simulink model "LunarMicrogrid_Full_Arch"  (R2026b)
settings: Solver=ode23t  StopTime=simulation.timeSim  MaxStep=1/(5*solarPlant.converterSwitchingFrequency)  AbsTol=1e-3
PreLoadFcn:
  | run('LunarMicrogridA_Data');
values from neighbouring files (symbols this model uses):
  Csc = Csc_cell/Ns_sc*Np_sc    (= 200)    [LunarDAB_Params.m]
  eta_sc = 0.95    [LunarDAB_Params.m]
  fsw = 100e3    (= 100000)    [LunarDAB_Params.m]
  k_restore = 1    [LunarDAB_Params.m]
  kiCurrent = 2    [LunarDAB_Params.m]
  kiVoltage = 8    [LunarDAB_Params.m]
  kpCurrent = 0.005    [LunarDAB_Params.m]
  kpVoltage = 0.4    [LunarDAB_Params.m]
  lTotal = lSeries + Llk    [LunarDAB_Params.m]
  P170_dt = 1e-4    (= 0.0001)    [P170_PV_Initialize.m]
  P170_Imp = im(ix)    [P170_PV_Initialize.m]
  P170_Vmp = vm(ix)    [P170_PV_Initialize.m]
  Rd_bat = dV_droop/Ibat_max    (= 0.232258064516)    [LunarDAB_Params.m]
  SC_enable = 1    [LunarDAB_Params.m]
  thetaIC = 0    [LunarDAB_Params.m]
  thetaMaxDab = pi/4    (= 0.785398163397)    [LunarDAB_Params.m]
  Tsw = 1/fsw    (= 1e-05)    [LunarDAB_Params.m]
  Vsc0 = sqrt((Vsc_max^2 + Vsc_min^2)/2)    [LunarDAB_Params.m]
  Vsc_max = 119    [LunarDAB_Params.m]
  Vsc_min = 66    [LunarDAB_Params.m]
undefined symbols (not defined in the file or in its folder): a_lpf_sys, battery, bms, connectedLoad, dcVoltage, DiscIntNeverNeededParam, eta_dab, Ibat_sign, mmc, Ndab, P170_T, pvDroop, sc, sensor, socLimit, solarPlant
libraries: sl_discontinuities x13, fl_lib x13, nesl_utility x13, simulink x7, batteryecm_lib x1, simulink_extras x1, ee_lib x1
(part 8 of 8)

== system LunarMicrogrid_Full_Arch/Battery + DAB + Supercap/BESS Controller/PIctrl/Anti-windup/Disc. Clamping Ideal/Dead Zone ==
  preSat : Inport
  Upper Limit : Inport  Port=2  SampleTime=SampleTime
  Lower Limit : Inport  Port=3  SampleTime=SampleTime
  Disabled : Subsystem  VariantControl=Disabled
  Enabled : Subsystem  VariantControl=Enabled
  External : Subsystem  VariantControl=External
  DZ out : Outport

== system LunarMicrogrid_Full_Arch/Battery + DAB + Supercap/BESS Controller/PIctrl/Anti-windup/Disc. Clamping Parallel/Dead Zone ==
  preSat : Inport
  Upper Limit : Inport  Port=2  SampleTime=SampleTime
  Lower Limit : Inport  Port=3  SampleTime=SampleTime
  Disabled : Subsystem  VariantControl=Disabled
  Enabled : Subsystem  VariantControl=Enabled
  External : Subsystem  VariantControl=External
  DZ out : Outport

== system LunarMicrogrid_Full_Arch/Battery + DAB + Supercap/BESS Controller/PIctrl/Filter/Differentiator/Tsamp ==
  U : Inport  SampleTime=SampleTime
  Ts : Inport  Port=2  SampleTime=SampleTime
  External Ts : Subsystem  VariantControl=ExternalTs
  Internal Ts : Subsystem  VariantControl=InternalTs
  Out1 : Outport  SampleTime=SampleTime

== system LunarMicrogrid_Full_Arch/Battery + DAB + Supercap/BESS Controller/PIctrl/Filter/Disc. Backward Euler Filter/Tsamp ==
  N : Inport  SampleTime=SampleTime
  Ts : Inport  Port=2  SampleTime=SampleTime
  External Ts : Subsystem  VariantControl=ExternalTs
  Internal Ts : Subsystem  VariantControl=InternalTs
  Out1 : Outport  SampleTime=SampleTime

== system LunarMicrogrid_Full_Arch/Battery + DAB + Supercap/BESS Controller/PIctrl/Filter/Disc. Backward Euler Filter Only/Tsamp ==
  N : Inport  SampleTime=SampleTime
  Ts : Inport  Port=2  SampleTime=SampleTime
  External Ts : Subsystem  VariantControl=ExternalTs
  Internal Ts : Subsystem  VariantControl=InternalTs
  Out1 : Outport  SampleTime=SampleTime

== system LunarMicrogrid_Full_Arch/Battery + DAB + Supercap/BESS Controller/PIctrl/Filter/Disc. Trapezoidal Filter/Tsamp ==
  N : Inport  SampleTime=SampleTime
  Ts : Inport  Port=2  SampleTime=SampleTime
  External Ts : Subsystem  VariantControl=ExternalTs
  Internal Ts : Subsystem  VariantControl=InternalTs
  Out1 : Outport  SampleTime=SampleTime

== system LunarMicrogrid_Full_Arch/Battery + DAB + Supercap/BESS Controller/PIctrl/Filter/Disc. Trapezoidal Filter Only/Tsamp ==
  N : Inport  SampleTime=SampleTime
  Ts : Inport  Port=2  SampleTime=SampleTime
  External Ts : Subsystem  VariantControl=ExternalTs
  Internal Ts : Subsystem  VariantControl=InternalTs
  Out1 : Outport  SampleTime=SampleTime

== system LunarMicrogrid_Full_Arch/Battery + DAB + Supercap/BESS Controller/DABCtrl2/Anti-windup/Cont. Clamping Ideal/Dead Zone/Disabled ==

== system LunarMicrogrid_Full_Arch/Battery + DAB + Supercap/BESS Controller/DABCtrl2/Anti-windup/Cont. Clamping Ideal/Dead Zone/Enabled ==
  preSat : Inport
  DeadZone : DeadZone  DisableCoverage=on  LowerValue=LowerSaturationLimit  UpperValue=UpperSaturationLimit  LinearizeAsGain=off  SaturateOnIntegerOverflow=off
  DZ out : Outport
  wires:
  preSat/1 -> DeadZone/1
  DeadZone/1 -> DZ out/1

== system LunarMicrogrid_Full_Arch/Battery + DAB + Supercap/BESS Controller/DABCtrl2/Anti-windup/Cont. Clamping Ideal/Dead Zone/External ==
  preSat : Inport
  Upper Limit : Inport  Port=2  SampleTime=SampleTime
  Lower Limit : Inport  Port=3  SampleTime=SampleTime
  Dead Zone Dynamic1 : sl_discontinuities/Dead Zone Dynamic
  DZ out : Outport
  wires:
  preSat/1 -> Dead Zone Dynamic1/2
  Lower Limit/1 -> Dead Zone Dynamic1/3
  Upper Limit/1 -> Dead Zone Dynamic1/1
  Dead Zone Dynamic1/1 -> DZ out/1

== system LunarMicrogrid_Full_Arch/Battery + DAB + Supercap/BESS Controller/DABCtrl2/Anti-windup/Cont. Clamping Parallel/Dead Zone/Disabled ==

== system LunarMicrogrid_Full_Arch/Battery + DAB + Supercap/BESS Controller/DABCtrl2/Anti-windup/Cont. Clamping Parallel/Dead Zone/Enabled ==
  preSat : Inport
  DeadZone : DeadZone  DisableCoverage=on  LowerValue=LowerSaturationLimit  UpperValue=UpperSaturationLimit  LinearizeAsGain=off  SaturateOnIntegerOverflow=off
  DZ out : Outport
  wires:
  preSat/1 -> DeadZone/1
  DeadZone/1 -> DZ out/1

== system LunarMicrogrid_Full_Arch/Battery + DAB + Supercap/BESS Controller/DABCtrl2/Anti-windup/Cont. Clamping Parallel/Dead Zone/External ==
  preSat : Inport
  Upper Limit : Inport  Port=2  SampleTime=SampleTime
  Lower Limit : Inport  Port=3  SampleTime=SampleTime
  Dead Zone Dynamic : sl_discontinuities/Dead Zone Dynamic
  DZ out : Outport
  wires:
  preSat/1 -> Dead Zone Dynamic/2
  Lower Limit/1 -> Dead Zone Dynamic/3
  Upper Limit/1 -> Dead Zone Dynamic/1
  Dead Zone Dynamic/1 -> DZ out/1

== system LunarMicrogrid_Full_Arch/Battery + DAB + Supercap/BESS Controller/DABCtrl2/Anti-windup/Disc. Clamping Ideal/Dead Zone/Disabled ==

== system LunarMicrogrid_Full_Arch/Battery + DAB + Supercap/BESS Controller/DABCtrl2/Anti-windup/Disc. Clamping Ideal/Dead Zone/Enabled ==
  preSat : Inport
  DeadZone : DeadZone  DisableCoverage=on  LowerValue=LowerSaturationLimit  UpperValue=UpperSaturationLimit  LinearizeAsGain=off  SaturateOnIntegerOverflow=off
  DZ out : Outport
  wires:
  DeadZone/1 -> DZ out/1
  preSat/1 -> DeadZone/1

== system LunarMicrogrid_Full_Arch/Battery + DAB + Supercap/BESS Controller/DABCtrl2/Anti-windup/Disc. Clamping Ideal/Dead Zone/External ==
  preSat : Inport
  Upper Limit : Inport  Port=2  SampleTime=SampleTime
  Lower Limit : Inport  Port=3  SampleTime=SampleTime
  Dead Zone Dynamic : sl_discontinuities/Dead Zone Dynamic
  DZ out : Outport
  wires:
  Dead Zone Dynamic/1 -> DZ out/1
  Upper Limit/1 -> Dead Zone Dynamic/1
  Lower Limit/1 -> Dead Zone Dynamic/3
  preSat/1 -> Dead Zone Dynamic/2

== system LunarMicrogrid_Full_Arch/Battery + DAB + Supercap/BESS Controller/DABCtrl2/Anti-windup/Disc. Clamping Parallel/Dead Zone/Disabled ==

== system LunarMicrogrid_Full_Arch/Battery + DAB + Supercap/BESS Controller/DABCtrl2/Anti-windup/Disc. Clamping Parallel/Dead Zone/Enabled ==
  preSat : Inport
  DeadZone : DeadZone  DisableCoverage=on  LowerValue=LowerSaturationLimit  UpperValue=UpperSaturationLimit  LinearizeAsGain=off  SaturateOnIntegerOverflow=off
  DZ out : Outport
  wires:
  DeadZone/1 -> DZ out/1
  preSat/1 -> DeadZone/1

== system LunarMicrogrid_Full_Arch/Battery + DAB + Supercap/BESS Controller/DABCtrl2/Anti-windup/Disc. Clamping Parallel/Dead Zone/External ==
  preSat : Inport
  Upper Limit : Inport  Port=2  SampleTime=SampleTime
  Lower Limit : Inport  Port=3  SampleTime=SampleTime
  Dead Zone Dynamic : sl_discontinuities/Dead Zone Dynamic
  DZ out : Outport
  wires:
  Dead Zone Dynamic/1 -> DZ out/1
  Upper Limit/1 -> Dead Zone Dynamic/1
  Lower Limit/1 -> Dead Zone Dynamic/3
  preSat/1 -> Dead Zone Dynamic/2

== system LunarMicrogrid_Full_Arch/Battery + DAB + Supercap/BESS Controller/DABCtrl2/Filter/Differentiator/Tsamp/External Ts ==
  U : Inport  SampleTime=SampleTime
  Ts : Inport  Port=2  SampleTime=SampleTime
  Udiff*Ts Prod Out : Product  Inputs=*/  OutMin=UdiffTsProdOutMin  OutMax=UdiffTsProdOutMax  RndMeth=Simplest  SampleTime=SampleTime
  Out1 : Outport  SampleTime=SampleTime
  wires:
  U/1 -> Udiff*Ts Prod Out/1
  Udiff*Ts Prod Out/1 -> Out1/1
  Ts/1 -> Udiff*Ts Prod Out/2

== system LunarMicrogrid_Full_Arch/Battery + DAB + Supercap/BESS Controller/DABCtrl2/Filter/Differentiator/Tsamp/Internal Ts ==
  U : Inport  SampleTime=SampleTime
  Ts : Inport  Port=2  SampleTime=SampleTime
  Terminator : Terminator
  Tsamp : SampleTimeMath  TsampMathOp=/  TsampMathImp=Offline Scaling Adjustment  RndMeth=Simplest
  Out1 : Outport  SampleTime=SampleTime
  wires:
  U/1 -> Tsamp/1
  Ts/1 -> Terminator/1
  Tsamp/1 -> Out1/1

== system LunarMicrogrid_Full_Arch/Battery + DAB + Supercap/BESS Controller/DABCtrl2/Filter/Disc. Backward Euler Filter/Tsamp/External Ts ==
  N : Inport  SampleTime=SampleTime
  Ts : Inport  Port=2  SampleTime=SampleTime
  N*Ts Prod Out : Product  OutMin=NTsProdOutMin  OutMax=NTsProdOutMax  RndMeth=Simplest  SampleTime=SampleTime
  Out1 : Outport  SampleTime=SampleTime
  wires:
  Ts/1 -> N*Ts Prod Out/2
  N*Ts Prod Out/1 -> Out1/1
  N/1 -> N*Ts Prod Out/1

== system LunarMicrogrid_Full_Arch/Battery + DAB + Supercap/BESS Controller/DABCtrl2/Filter/Disc. Backward Euler Filter/Tsamp/Internal Ts ==
  N : Inport  SampleTime=SampleTime
  Ts : Inport  Port=2  SampleTime=SampleTime
  Terminator : Terminator
  Tsamp : SampleTimeMath  TsampMathOp=*  RndMeth=Simplest
  Out1 : Outport  SampleTime=SampleTime
  wires:
  Tsamp/1 -> Out1/1
  Ts/1 -> Terminator/1
  N/1 -> Tsamp/1

== system LunarMicrogrid_Full_Arch/Battery + DAB + Supercap/BESS Controller/DABCtrl2/Filter/Disc. Backward Euler Filter Only/Tsamp/External Ts ==
  N : Inport  SampleTime=SampleTime
  Ts : Inport  Port=2  SampleTime=SampleTime
  N*Ts Prod Out : Product  OutMin=NTsProdOutMin  OutMax=NTsProdOutMax  SampleTime=SampleTime
  Out1 : Outport  SampleTime=SampleTime
  wires:
  N/1 -> N*Ts Prod Out/1
  N*Ts Prod Out/1 -> Out1/1
  Ts/1 -> N*Ts Prod Out/2

== system LunarMicrogrid_Full_Arch/Battery + DAB + Supercap/BESS Controller/DABCtrl2/Filter/Disc. Backward Euler Filter Only/Tsamp/Internal Ts ==
  N : Inport  SampleTime=SampleTime
  Ts : Inport  Port=2  SampleTime=SampleTime
  Terminator : Terminator
  Tsamp : SampleTimeMath  TsampMathOp=*
  Out1 : Outport  SampleTime=SampleTime
  wires:
  N/1 -> Tsamp/1
  Ts/1 -> Terminator/1
  Tsamp/1 -> Out1/1

== system LunarMicrogrid_Full_Arch/Battery + DAB + Supercap/BESS Controller/DABCtrl2/Filter/Disc. Trapezoidal Filter/Tsamp/External Ts ==
  N : Inport  SampleTime=SampleTime
  Ts : Inport  Port=2  SampleTime=SampleTime
  Gain : Gain  Gain=0.5  RndMeth=Simplest
  N*Ts Prod Out : Product  OutMin=NTsProdOutMin  OutMax=NTsProdOutMax  RndMeth=Simplest  SampleTime=SampleTime
  Out1 : Outport  SampleTime=SampleTime
  wires:
  Gain/1 -> N*Ts Prod Out/2
  Ts/1 -> Gain/1
  N*Ts Prod Out/1 -> Out1/1
  N/1 -> N*Ts Prod Out/1

== system LunarMicrogrid_Full_Arch/Battery + DAB + Supercap/BESS Controller/DABCtrl2/Filter/Disc. Trapezoidal Filter/Tsamp/Internal Ts ==
  N : Inport  SampleTime=SampleTime
  Ts : Inport  Port=2  SampleTime=SampleTime
  Terminator : Terminator
  Tsamp : SampleTimeMath  TsampMathOp=*  weightValue=0.5  RndMeth=Simplest
  Out1 : Outport  SampleTime=SampleTime
  wires:
  Tsamp/1 -> Out1/1
  Ts/1 -> Terminator/1
  N/1 -> Tsamp/1

== system LunarMicrogrid_Full_Arch/Battery + DAB + Supercap/BESS Controller/DABCtrl2/Filter/Disc. Trapezoidal Filter Only/Tsamp/External Ts ==
  N : Inport  SampleTime=SampleTime
  Ts : Inport  Port=2  SampleTime=SampleTime
  Gain : Gain  Gain=0.5
  N*Ts Prod Out : Product  OutMin=NTsProdOutMin  OutMax=NTsProdOutMax  SampleTime=SampleTime
  Out1 : Outport  SampleTime=SampleTime
  wires:
  N/1 -> N*Ts Prod Out/1
  N*Ts Prod Out/1 -> Out1/1
  Ts/1 -> Gain/1
  Gain/1 -> N*Ts Prod Out/2

== system LunarMicrogrid_Full_Arch/Battery + DAB + Supercap/BESS Controller/DABCtrl2/Filter/Disc. Trapezoidal Filter Only/Tsamp/Internal Ts ==
  N : Inport  SampleTime=SampleTime
  Ts : Inport  Port=2  SampleTime=SampleTime
  Terminator : Terminator
  Tsamp : SampleTimeMath  TsampMathOp=*  weightValue=0.5
  Out1 : Outport  SampleTime=SampleTime
  wires:
  N/1 -> Tsamp/1
  Ts/1 -> Terminator/1
  Tsamp/1 -> Out1/1

== system LunarMicrogrid_Full_Arch/Battery + DAB + Supercap/BESS Controller/PIctrl/Anti-windup/Cont. Clamping Ideal/Dead Zone/Disabled ==

== system LunarMicrogrid_Full_Arch/Battery + DAB + Supercap/BESS Controller/PIctrl/Anti-windup/Cont. Clamping Ideal/Dead Zone/Enabled ==
  preSat : Inport
  DeadZone : DeadZone  DisableCoverage=on  LowerValue=LowerSaturationLimit  UpperValue=UpperSaturationLimit  LinearizeAsGain=off  SaturateOnIntegerOverflow=off
  DZ out : Outport
  wires:
  preSat/1 -> DeadZone/1
  DeadZone/1 -> DZ out/1

== system LunarMicrogrid_Full_Arch/Battery + DAB + Supercap/BESS Controller/PIctrl/Anti-windup/Cont. Clamping Ideal/Dead Zone/External ==
  preSat : Inport
  Upper Limit : Inport  Port=2  SampleTime=SampleTime
  Lower Limit : Inport  Port=3  SampleTime=SampleTime
  Dead Zone Dynamic1 : sl_discontinuities/Dead Zone Dynamic
  DZ out : Outport
  wires:
  preSat/1 -> Dead Zone Dynamic1/2
  Lower Limit/1 -> Dead Zone Dynamic1/3
  Upper Limit/1 -> Dead Zone Dynamic1/1
  Dead Zone Dynamic1/1 -> DZ out/1

== system LunarMicrogrid_Full_Arch/Battery + DAB + Supercap/BESS Controller/PIctrl/Anti-windup/Cont. Clamping Parallel/Dead Zone/Disabled ==

== system LunarMicrogrid_Full_Arch/Battery + DAB + Supercap/BESS Controller/PIctrl/Anti-windup/Cont. Clamping Parallel/Dead Zone/Enabled ==
  preSat : Inport
  DeadZone : DeadZone  DisableCoverage=on  LowerValue=LowerSaturationLimit  UpperValue=UpperSaturationLimit  LinearizeAsGain=off  SaturateOnIntegerOverflow=off
  DZ out : Outport
  wires:
  preSat/1 -> DeadZone/1
  DeadZone/1 -> DZ out/1

== system LunarMicrogrid_Full_Arch/Battery + DAB + Supercap/BESS Controller/PIctrl/Anti-windup/Cont. Clamping Parallel/Dead Zone/External ==
  preSat : Inport
  Upper Limit : Inport  Port=2  SampleTime=SampleTime
  Lower Limit : Inport  Port=3  SampleTime=SampleTime
  Dead Zone Dynamic : sl_discontinuities/Dead Zone Dynamic
  DZ out : Outport
  wires:
  preSat/1 -> Dead Zone Dynamic/2
  Lower Limit/1 -> Dead Zone Dynamic/3
  Upper Limit/1 -> Dead Zone Dynamic/1
  Dead Zone Dynamic/1 -> DZ out/1

== system LunarMicrogrid_Full_Arch/Battery + DAB + Supercap/BESS Controller/PIctrl/Anti-windup/Disc. Clamping Ideal/Dead Zone/Disabled ==

== system LunarMicrogrid_Full_Arch/Battery + DAB + Supercap/BESS Controller/PIctrl/Anti-windup/Disc. Clamping Ideal/Dead Zone/Enabled ==
  preSat : Inport
  DeadZone : DeadZone  DisableCoverage=on  LowerValue=LowerSaturationLimit  UpperValue=UpperSaturationLimit  LinearizeAsGain=off  SaturateOnIntegerOverflow=off
  DZ out : Outport
  wires:
  DeadZone/1 -> DZ out/1
  preSat/1 -> DeadZone/1

== system LunarMicrogrid_Full_Arch/Battery + DAB + Supercap/BESS Controller/PIctrl/Anti-windup/Disc. Clamping Ideal/Dead Zone/External ==
  preSat : Inport
  Upper Limit : Inport  Port=2  SampleTime=SampleTime
  Lower Limit : Inport  Port=3  SampleTime=SampleTime
  Dead Zone Dynamic : sl_discontinuities/Dead Zone Dynamic
  DZ out : Outport
  wires:
  Dead Zone Dynamic/1 -> DZ out/1
  Upper Limit/1 -> Dead Zone Dynamic/1
  Lower Limit/1 -> Dead Zone Dynamic/3
  preSat/1 -> Dead Zone Dynamic/2

== system LunarMicrogrid_Full_Arch/Battery + DAB + Supercap/BESS Controller/PIctrl/Anti-windup/Disc. Clamping Parallel/Dead Zone/Disabled ==

== system LunarMicrogrid_Full_Arch/Battery + DAB + Supercap/BESS Controller/PIctrl/Anti-windup/Disc. Clamping Parallel/Dead Zone/Enabled ==
  preSat : Inport
  DeadZone : DeadZone  DisableCoverage=on  LowerValue=LowerSaturationLimit  UpperValue=UpperSaturationLimit  LinearizeAsGain=off  SaturateOnIntegerOverflow=off
  DZ out : Outport
  wires:
  DeadZone/1 -> DZ out/1
  preSat/1 -> DeadZone/1

== system LunarMicrogrid_Full_Arch/Battery + DAB + Supercap/BESS Controller/PIctrl/Anti-windup/Disc. Clamping Parallel/Dead Zone/External ==
  preSat : Inport
  Upper Limit : Inport  Port=2  SampleTime=SampleTime
  Lower Limit : Inport  Port=3  SampleTime=SampleTime
  Dead Zone Dynamic : sl_discontinuities/Dead Zone Dynamic
  DZ out : Outport
  wires:
  Dead Zone Dynamic/1 -> DZ out/1
  Upper Limit/1 -> Dead Zone Dynamic/1
  Lower Limit/1 -> Dead Zone Dynamic/3
  preSat/1 -> Dead Zone Dynamic/2

== system LunarMicrogrid_Full_Arch/Battery + DAB + Supercap/BESS Controller/PIctrl/Filter/Differentiator/Tsamp/External Ts ==
  U : Inport  SampleTime=SampleTime
  Ts : Inport  Port=2  SampleTime=SampleTime
  Udiff*Ts Prod Out : Product  Inputs=*/  OutMin=UdiffTsProdOutMin  OutMax=UdiffTsProdOutMax  RndMeth=Simplest  SampleTime=SampleTime
  Out1 : Outport  SampleTime=SampleTime
  wires:
  U/1 -> Udiff*Ts Prod Out/1
  Udiff*Ts Prod Out/1 -> Out1/1
  Ts/1 -> Udiff*Ts Prod Out/2

== system LunarMicrogrid_Full_Arch/Battery + DAB + Supercap/BESS Controller/PIctrl/Filter/Differentiator/Tsamp/Internal Ts ==
  U : Inport  SampleTime=SampleTime
  Ts : Inport  Port=2  SampleTime=SampleTime
  Terminator : Terminator
  Tsamp : SampleTimeMath  TsampMathOp=/  TsampMathImp=Offline Scaling Adjustment  RndMeth=Simplest
  Out1 : Outport  SampleTime=SampleTime
  wires:
  U/1 -> Tsamp/1
  Ts/1 -> Terminator/1
  Tsamp/1 -> Out1/1

== system LunarMicrogrid_Full_Arch/Battery + DAB + Supercap/BESS Controller/PIctrl/Filter/Disc. Backward Euler Filter/Tsamp/External Ts ==
  N : Inport  SampleTime=SampleTime
  Ts : Inport  Port=2  SampleTime=SampleTime
  N*Ts Prod Out : Product  OutMin=NTsProdOutMin  OutMax=NTsProdOutMax  RndMeth=Simplest  SampleTime=SampleTime
  Out1 : Outport  SampleTime=SampleTime
  wires:
  Ts/1 -> N*Ts Prod Out/2
  N*Ts Prod Out/1 -> Out1/1
  N/1 -> N*Ts Prod Out/1

== system LunarMicrogrid_Full_Arch/Battery + DAB + Supercap/BESS Controller/PIctrl/Filter/Disc. Backward Euler Filter/Tsamp/Internal Ts ==
  N : Inport  SampleTime=SampleTime
  Ts : Inport  Port=2  SampleTime=SampleTime
  Terminator : Terminator
  Tsamp : SampleTimeMath  TsampMathOp=*  RndMeth=Simplest
  Out1 : Outport  SampleTime=SampleTime
  wires:
  Tsamp/1 -> Out1/1
  Ts/1 -> Terminator/1
  N/1 -> Tsamp/1

== system LunarMicrogrid_Full_Arch/Battery + DAB + Supercap/BESS Controller/PIctrl/Filter/Disc. Backward Euler Filter Only/Tsamp/External Ts ==
  N : Inport  SampleTime=SampleTime
  Ts : Inport  Port=2  SampleTime=SampleTime
  N*Ts Prod Out : Product  OutMin=NTsProdOutMin  OutMax=NTsProdOutMax  SampleTime=SampleTime
  Out1 : Outport  SampleTime=SampleTime
  wires:
  N/1 -> N*Ts Prod Out/1
  N*Ts Prod Out/1 -> Out1/1
  Ts/1 -> N*Ts Prod Out/2

== system LunarMicrogrid_Full_Arch/Battery + DAB + Supercap/BESS Controller/PIctrl/Filter/Disc. Backward Euler Filter Only/Tsamp/Internal Ts ==
  N : Inport  SampleTime=SampleTime
  Ts : Inport  Port=2  SampleTime=SampleTime
  Terminator : Terminator
  Tsamp : SampleTimeMath  TsampMathOp=*
  Out1 : Outport  SampleTime=SampleTime
  wires:
  N/1 -> Tsamp/1
  Ts/1 -> Terminator/1
  Tsamp/1 -> Out1/1

== system LunarMicrogrid_Full_Arch/Battery + DAB + Supercap/BESS Controller/PIctrl/Filter/Disc. Trapezoidal Filter/Tsamp/External Ts ==
  N : Inport  SampleTime=SampleTime
  Ts : Inport  Port=2  SampleTime=SampleTime
  Gain : Gain  Gain=0.5  RndMeth=Simplest
  N*Ts Prod Out : Product  OutMin=NTsProdOutMin  OutMax=NTsProdOutMax  RndMeth=Simplest  SampleTime=SampleTime
  Out1 : Outport  SampleTime=SampleTime
  wires:
  Gain/1 -> N*Ts Prod Out/2
  Ts/1 -> Gain/1
  N*Ts Prod Out/1 -> Out1/1
  N/1 -> N*Ts Prod Out/1

== system LunarMicrogrid_Full_Arch/Battery + DAB + Supercap/BESS Controller/PIctrl/Filter/Disc. Trapezoidal Filter/Tsamp/Internal Ts ==
  N : Inport  SampleTime=SampleTime
  Ts : Inport  Port=2  SampleTime=SampleTime
  Terminator : Terminator
  Tsamp : SampleTimeMath  TsampMathOp=*  weightValue=0.5  RndMeth=Simplest
  Out1 : Outport  SampleTime=SampleTime
  wires:
  Tsamp/1 -> Out1/1
  Ts/1 -> Terminator/1
  N/1 -> Tsamp/1

== system LunarMicrogrid_Full_Arch/Battery + DAB + Supercap/BESS Controller/PIctrl/Filter/Disc. Trapezoidal Filter Only/Tsamp/External Ts ==
  N : Inport  SampleTime=SampleTime
  Ts : Inport  Port=2  SampleTime=SampleTime
  Gain : Gain  Gain=0.5
  N*Ts Prod Out : Product  OutMin=NTsProdOutMin  OutMax=NTsProdOutMax  SampleTime=SampleTime
  Out1 : Outport  SampleTime=SampleTime
  wires:
  N/1 -> N*Ts Prod Out/1
  N*Ts Prod Out/1 -> Out1/1
  Ts/1 -> Gain/1
  Gain/1 -> N*Ts Prod Out/2

== system LunarMicrogrid_Full_Arch/Battery + DAB + Supercap/BESS Controller/PIctrl/Filter/Disc. Trapezoidal Filter Only/Tsamp/Internal Ts ==
  N : Inport  SampleTime=SampleTime
  Ts : Inport  Port=2  SampleTime=SampleTime
  Terminator : Terminator
  Tsamp : SampleTimeMath  TsampMathOp=*  weightValue=0.5
  Out1 : Outport  SampleTime=SampleTime
  wires:
  N/1 -> Tsamp/1
  Ts/1 -> Terminator/1
  Tsamp/1 -> Out1/1

== matlab function LunarMicrogrid_Full_Arch/MMC Intertie to Site B (1.5 kV)/MMC Intertie ==
  settings: updateMethod=DISCRETE  sampleTime=mmc.dt
  data: Vbus input; I_LV output; P_rx input; P output; V_HV output; I_line output; V_rx output; phi output; mmc parameter
function [I_LV, P, V_HV, I_line, V_rx, phi] = fcn(Vbus, P_rx, mmc)
% averaged MMC intertie, same equations as mmc_and_bus_current.m
% uses the real 120 V bus voltage instead of a fixed 120 V
persistent V I Vrx z
if isempty(V)
    V = mmc.V0; I = mmc.I0; Vrx = mmc.Vrx0; z = mmc.z0;
end
dt = mmc.dt;
vb = max(Vbus, 1);
e = mmc.V_ref - V;
u = mmc.Kp*e + mmc.Ki*z;
phi = min(max(u, -pi/2), pi/2);
if ~((u >= pi/2 && e > 0) || (u <= -pi/2 && e < 0)), z = z + e*dt; end
Kc = mmc.n*vb*V/(2*pi*mmc.rv*mmc.f*mmc.Lleak);
P = mmc.Npar*Kc*phi*(1 - abs(phi)/pi);
dV  = (P/V - I)/mmc.C_HV;
dI  = (V - Vrx - mmc.R_line*I)/mmc.L_line;
dVr = (I - P_rx/max(Vrx, 1))/mmc.C_RX;
V_HV = V; I_line = I; V_rx = Vrx;
V = V + dV*dt; I = I + dI*dt; Vrx = Vrx + dVr*dt;
I_LV = P/vb;
end

== matlab function LunarMicrogrid_Full_Arch/PV Array + Converter/PV_MPPT_6module ==
  settings: updateMethod=DISCRETE  sampleTime=P170_dt
  data: G input; Ibus output; T input; Vbus input; en input; VmpT input; ImpT input; Pbus output; Pavail output; Vpv output; Ipv output; Imod output; duty output
function [Ibus, Pbus, Pavail, Vpv, Ipv, Imod, duty] = fcn(G,T,Vbus,en,VmpT,ImpT)
%#codegen
% EOL teammate MPP data; illustrative piecewise I-V fit.
% Shared PV bus, single coordinated P&O, six averaged PI branches.
persistent Vcmd dir Pprev count il integ
if isempty(Vcmd)
 Vcmd=217; dir=1; Pprev=0; count=0; il=zeros(6,1); integ=zeros(6,1);
end
dt=1e-4; eta=0.96; Gref=1367;
gs=max(0,min(1.5,G/Gref));
vmp=max(10,VmpT); imp=max(0,ImpT)*gs;
% Curve passes through Isc, Imp at Vmp, and zero at Voc.
% Isc=1.04 Imp, Voc=1.13 Vmp are MODEL ASSUMPTIONS.
isc=1.04*imp; voc=1.13*vmp;
Vcmd=max(0.5*vmp,min(0.99*voc,Vcmd));
if Vcmd<=vmp
 ipv=max(0,isc-(isc-imp)*(Vcmd/vmp)^2);
else
 ipv=max(0,imp*(voc-Vcmd)/(voc-vmp));
end
Ppv=Vcmd*ipv; Pavail=max(0,vmp*imp*eta);
count=count+1;
if count>=100
 if Ppv<Pprev, dir=-dir; end
 Vcmd=Vcmd+dir*0.5; Pprev=Ppv; count=0;
end
% Power-to-current reference; current limited by PV production.
v=max(30,Vbus);
Ptarget=max(0,min(Ppv*eta,Pavail))*max(0,min(1,en));
Iref=Ptarget/v/6;
Imod=zeros(6,1); duty=zeros(6,1);
for k=1:6
 % Averaged current PI with feedforward; shared-array duty proxy.
 err=Iref-il(k);
 dff=Vbus/max(1,1.15*Vcmd);
 d=max(0,min(0.85,dff+0.0015*err+integ(k)));
 % Average inductor dynamics; 33 uH each.
 next=il(k)+dt*(1.15*Vcmd*d-Vbus)/33e-6;
 % Avoid nonphysical reverse PV current.
 next=max(0,next);
 % Anti-windup: integrate only when unsaturated or correcting.
 if (d>0 && d<0.85) || (d<=0 && err>0) || (d>=0.85 && err<0)
  integ(k)=integ(k)+3*dt*err;
 end
 il(k)=next; Imod(k)=next; duty(k)=d;
end
% Conservation clamp: do not inject more power than PV can supply.
Iraw=sum(Imod); Ibus=min(Iraw,Ptarget/v);
Pbus=Ibus*max(0,Vbus); Vpv=Vcmd; Ipv=ipv;
end
